simulink model "AirDragValidation"  (R2026b)
settings: Solver=VariableStepAuto
values from neighbouring files (symbols this model uses):
  A_BN_in = [xB'; yB'; zB']    [ValidationAirDrag.m]
  A_surf = [Ly*Lz; Lx*Lz; Lx*Ly; Ly*Lz; Lx*Lz; Lx*Ly;            A_panel; A_panel; A_panel; A_panel]    [ValidationAirDrag.m]
  CD = CD0    (= 2.2)    [ValidationAirDrag.m]
  e = e0    (= 0.001)    [ValidationAirDrag.m]    (also in max_disturbance.m = 0.0011)
  n = sqrt(mu_earth/R^3)    [ValidationAirDrag.m]
  n_earth = n_earth0    (= 7.292115e-05)    [ValidationAirDrag.m]
  N_surf = [1 0 0; 0 1 0; 0 0 1; -1 0 0; 0 -1 0; 0 0 -1;            1 0 0; -1 0 0; 1 0 0; -1 0 0]    [ValidationAirDrag.m]
  R = R_earth + Altitude    (= 6946.2)    [ValidationAirDrag.m]
  r_CM_mat = repmat(r_CM,1,10)    [ValidationAirDrag.m]
  R_CP_geom = [Lx/2 0 0; 0 Ly/2 0; 0 0 Lz/2;              -Lx/2 0 0; 0 -Ly/2 0; 0 0 -Lz/2;               0 d_panel 0; 0 d_panel 0; 0 -d_panel 0; 0 -d_panel 0]'    [ValidationAirDrag.m]
  r_N_in = R_PQW_to_N*[r*cos(theta_in); r*sin(theta_in); 0]    [ValidationAirDrag.m]
  R_PQW_to_N = Q0    [ValidationAirDrag.m]
  rho = rho0    (= 1.315e-13)    [ValidationAirDrag.m]
  theta_in = deg2rad(45)    [ValidationAirDrag.m]
libraries: matrix_library x1
settings Model: Creator=39333  LastModifiedBy=39333

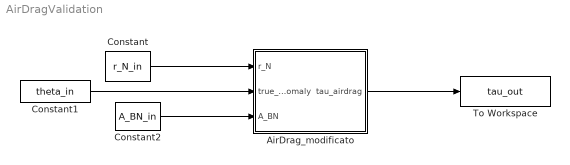
== system AirDragValidation ==
  AirDrag_modificato : Subsystem
  Constant : Constant  Value=r_N_in
  Constant1 : Constant  Value=theta_in
  Constant2 : Constant  Value=A_BN_in
  To Workspace : ToWorkspace  VariableName=tau_out  SaveFormat=Timeseries  SampleTime=-1
  wires:
  AirDrag_modificato/1(tau_airdrag) -> To Workspace/1
  Constant/1 -> AirDrag_modificato/1(r_N)
  Constant2/1 -> AirDrag_modificato/3(A_BN)
  Constant1/1 -> AirDrag_modificato/2(true_anomaly)

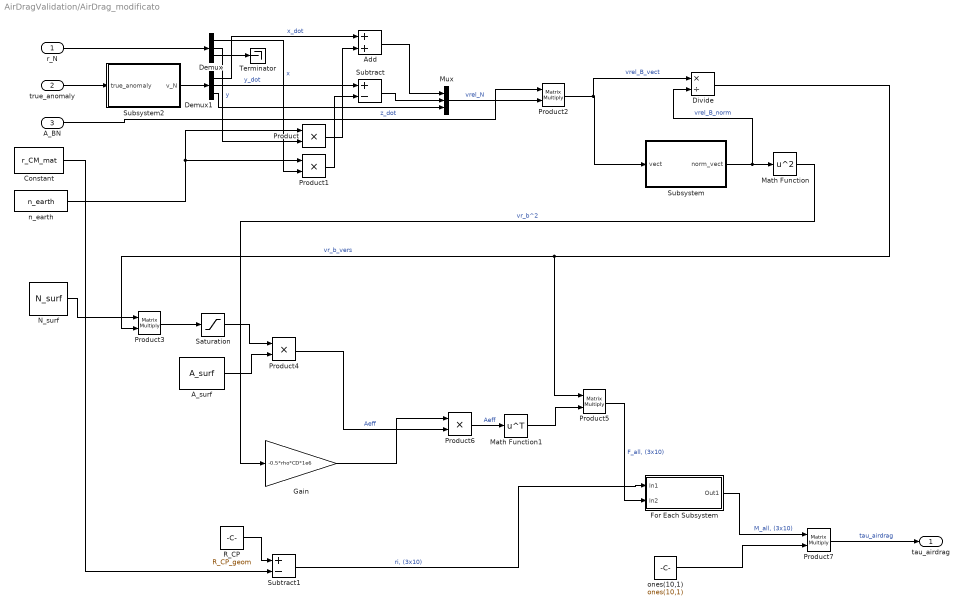
== system AirDragValidation/AirDrag_modificato ==
  r_N : Inport
  true_anomaly : Inport  Port=2
  A_BN : Inport  Port=3
  A_surf : Constant  Value=A_surf
  Add : Sum
  Constant : Constant  Value=r_CM_mat
  Demux : Demux  Outputs=3
  Demux1 : Demux  Outputs=3
  Divide : Product  Inputs=*/
  For Each Subsystem : Subsystem  TreatAsAtomicUnit=on
  Gain : Gain  Gain=-0.5*rho*CD*1e6
  Math Function : Math  Operator=square
  Math Function1 : Math  Operator=transpose
  Mux : Mux  Inputs=3
  N_surf : Constant  Value=N_surf
  Product{,1,4,6} (4 alike) : Product
  Product{2..3,5,7} (4 alike) : Product  Multiplication=Matrix(*)
  R_CP : Constant  Value=R_CP_geom
  Saturation : Saturate  UpperLimit=inf  LowerLimit=0
  Subsystem : Subsystem
  Subsystem2 : Subsystem
  Subtract : Sum  Inputs=+-
  Subtract1 : Sum  Inputs=+-
  Terminator : Terminator
  n_earth : Constant  Value=n_earth
  ones(10,1) : Constant  Value=ones(10,1)
  tau_airdrag : Outport
  wires:
  Divide/1 -> Product3/2, Product5/1  "vr_b_vers"
  Product4/1 -> Product6/2  "Aeff"
  n_earth/1 -> Product/1, Product1/1
  Demux/3 -> Terminator/1
  Math Function1/1 -> Product5/2
  Demux/2 -> Product/2  "y"
  Demux1/2 -> Subtract/1  "y_dot"
  Demux/1 -> Product1/2  "x"
  Product6/1 -> Math Function1/1  "Aeff"
  Product2/1 -> Divide/1, Subsystem/1(vect)  "vrel_B_vect"
  Gain/1 -> Product6/1
  Add/1 -> Mux/1
  For Each Subsystem/1(Out1) -> Product7/1  "M_all, (3x10)"
  Demux1/1 -> Add/1  "x_dot"
  Subsystem2/1(v_N) -> Demux1/1
  Subsystem/1(norm_vect) -> Divide/2, Math Function/1  "vrel_B_norm"
  A_surf/1 -> Product4/2
  Subtract/1 -> Mux/2
  R_CP/1 -> Subtract1/1
  Subtract1/1 -> For Each Subsystem/1(In1)  "ri, (3x10)"
  Demux1/3 -> Mux/3  "z_dot"
  Product/1 -> Add/2
  Mux/1 -> Product2/2  "vrel_N"
  Product3/1 -> Saturation/1
  Saturation/1 -> Product4/1
  A_BN/1 -> Product2/1
  Math Function/1 -> Gain/1  "vr_b^2"
  Product1/1 -> Subtract/2
  N_surf/1 -> Product3/1
  Product7/1 -> tau_airdrag/1  "tau_airdrag"
  ones(10,1)/1 -> Product7/2
  Product5/1 -> For Each Subsystem/2(In2)  "F_all, (3x10)"
  r_N/1 -> Demux/1
  true_anomaly/1 -> Subsystem2/1(true_anomaly)
  Constant/1 -> Subtract1/2

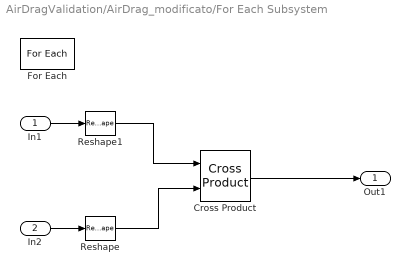
== system AirDragValidation/AirDrag_modificato/For Each Subsystem ==
  In1 : Inport  Partition=on  PartitionDimension=2  PartitionWidth=1  PartitionOffset=0
  In2 : Inport  Port=2  Partition=on  PartitionDimension=2  PartitionWidth=1  PartitionOffset=0
  Cross Product : matrix_library/Cross Product
  For Each : ForEach  DisableCoverage=on
  Reshape : Reshape
  Reshape1 : Reshape
  Out1 : Outport  ConcatenationDimension=2
  wires:
  Cross Product/1 -> Out1/1
  In2/1 -> Reshape/1
  In1/1 -> Reshape1/1
  Reshape1/1 -> Cross Product/1
  Reshape/1 -> Cross Product/2

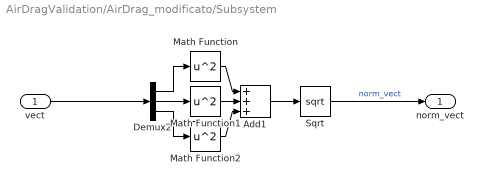
== system AirDragValidation/AirDrag_modificato/Subsystem ==
  vect : Inport
  Add1 : Sum  Inputs=+++
  Demux2 : Demux  Outputs=3
  Math Function : Math  Operator=square
  Math Function1 : Math  Operator=square
  Math Function2 : Math  Operator=square
  Sqrt : Sqrt
  norm_vect : Outport
  wires:
  Math Function1/1 -> Add1/2
  Math Function2/1 -> Add1/3
  Demux2/2 -> Math Function1/1
  Math Function/1 -> Add1/1
  vect/1 -> Demux2/1
  Demux2/3 -> Math Function2/1
  Demux2/1 -> Math Function/1
  Add1/1 -> Sqrt/1
  Sqrt/1 -> norm_vect/1  "norm_vect"

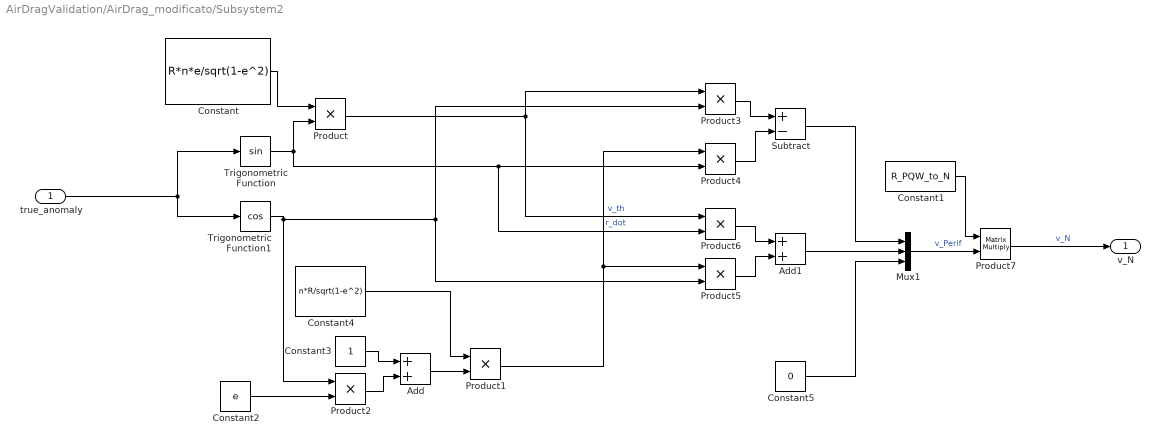
== system AirDragValidation/AirDrag_modificato/Subsystem2 ==
  true_anomaly : Inport
  Add : Sum
  Add1 : Sum
  Constant : Constant  Value=R*n*e/sqrt(1-e^2)
  Constant1 : Constant  Value=R_PQW_to_N
  Constant2 : Constant  Value=e
  Constant3 : Constant
  Constant4 : Constant  Value=n*R/sqrt(1-e^2)
  Constant5 : Constant  Value=0
  Mux1 : Mux  Inputs=3
  Product{,1..6} (7 alike) : Product
  Product7 : Product  Multiplication=Matrix(*)
  Subtract : Sum  Inputs=+-
  Trigonometric Function : Trigonometry
  Trigonometric Function1 : Trigonometry  Operator=cos
  v_N : Outport
  wires:
  Constant/1 -> Product/1
  Product1/1 -> Product4/1, Product5/1  "v_th"
  Trigonometric Function/1 -> Product6/2, Product4/2, Product/2
  Trigonometric Function1/1 -> Product3/2, Product5/2, Product2/1
  true_anomaly/1 -> Trigonometric Function/1, Trigonometric Function1/1
  Product2/1 -> Add/2
  Product/1 -> Product3/1, Product6/1  "r_dot"
  Constant4/1 -> Product1/1
  Constant2/1 -> Product2/2
  Add/1 -> Product1/2
  Constant3/1 -> Add/1
  Product7/1 -> v_N/1  "v_N"
  Product3/1 -> Subtract/1
  Product4/1 -> Subtract/2
  Product6/1 -> Add1/1
  Product5/1 -> Add1/2
  Add1/1 -> Mux1/2
  Subtract/1 -> Mux1/1
  Constant5/1 -> Mux1/3
  Mux1/1 -> Product7/2  "v_Perif"
  Constant1/1 -> Product7/1
